simulink model "aero2_position_integral"  (R2024b)
settings: Solver=ode1  StartTime=0.0  StopTime=60  FixedStep=0.002  RelTol=1e-3
model workspace (MAT data in the model file):
  Dpos = 5.83392170192
  Dq = 3.88928113461
  Kaw = 20
  Kff = 1
  Ki = 1.84164606325
  Kint = 7.35390515018
  Kp = 0.216370391856
  Kpos = 11.344880808
  Kq = 3.78162693601
  Kref = 3.78162693601
  ReferenceRate = [0 0.002 0.004 0.006 0.008 0.01 0.012 0.014 0.016 0.018 0.02 0.022 ... (90003 elements, 30001x3)]
  U_h = timeseries
  U_h.Name = 'unnamed'
  U_h.DataInfo = tsdata.datametadata
  U_h.DataInfo.Interpolation = tsdata.interpolation
  U_h.DataInfo.Interpolation.Fhandle : function handle (value not decoded)
  U_h.DataInfo.Interpolation.Name = 'linear'
  U_h.TimeInfo = tsdata.timemetadata
  U_h.TimeInfo.Length = 30001
  U_h.TimeInfo.DuplicateTimes = 0
  U_h.TimeInfo.Time_ = [0 0.002 0.004 0.006 0.008 0.01 0.012 0.014 0.016 0.018 0.02 0.022 ... (30001 elements, 30001x1)]
  U_h.TimeInfo.Initialized = 1
  U_h.QualityInfo = tsdata.qualmetadata
  U_h.Data_ = [0 0 0 0 0 0 0 0 0 0 0 0 ... (30001 elements, 30001x1)]
  U_v = timeseries
  U_v.Name = 'unnamed'
  U_v.DataInfo = tsdata.datametadata
  U_v.DataInfo.Interpolation = tsdata.interpolation
  U_v.DataInfo.Interpolation.Fhandle : function handle (value not decoded)
  U_v.DataInfo.Interpolation.Name = 'linear'
  U_v.TimeInfo = tsdata.timemetadata
  U_v.TimeInfo.Length = 30001
  U_v.TimeInfo.DuplicateTimes = 0
  U_v.TimeInfo.Time_ = [0 0.002 0.004 0.006 0.008 0.01 0.012 0.014 0.016 0.018 0.02 0.022 ... (30001 elements, 30001x1)]
  U_v.TimeInfo.Initialized = 1
  U_v.QualityInfo = tsdata.qualmetadata
  U_v.Data_ = [0 0 0 0 0 0 0 0 0 0 0 0 ... (30001 elements, 30001x1)]
  X0 = [0; 0; 0; 0]
  meas_on = 0
(part 1 of 2)
settings Model: Creator=matiasgarcia  LastModifiedBy=matiasgarcia
settings DataIOCC: SaveOutput=off  SignalLogging=off  SaveTime=off

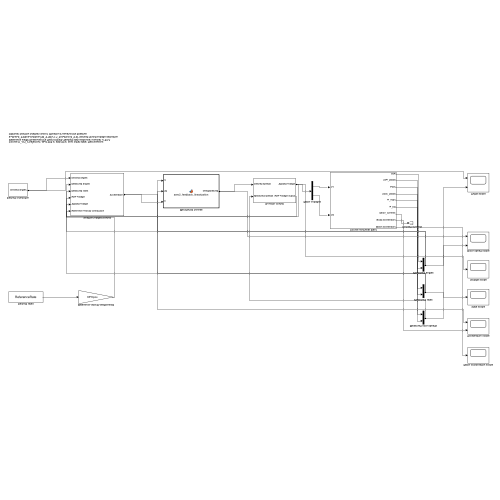
[thumbnail: Simulink's stored preview of the top-level diagram]
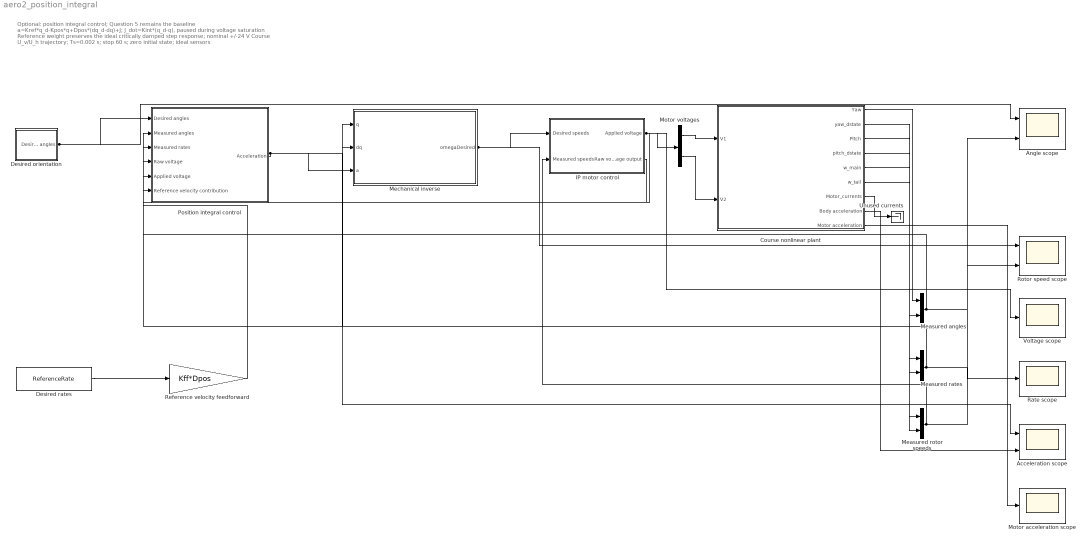
== system aero2_position_integral ==
  note: Optional: position integral control; Question 5 remains the baseline
      | a=Kref*q_d-Kpos*q+Dpos*(dq_d-dq)+J; J_dot=Kint*(q_d-q), paused during voltage saturation
      | Reference weight preserves the ideal critically damped step response; nominal +/-24 V
      | Course U_v/U_h trajectory; Ts=0.002 s; stop 60 s; zero initial state; ideal sensors
  Acceleration scope : Scope  NumInputPorts=2
  Angle scope : Scope  NumInputPorts=2
  Course nonlinear plant : Subsystem  mask{meas=meas_on}
      mask prompts: meas "Measurement effects (1 = encoder quantization + sensor noise, 0 = ideal)"
      mask help: Simplified twin-rotor model (eq. (simp) of twin_rotor_FL_merged.tex) with DC-motor rotor dynamics. Inputs: V1 main-rotor voltage, V2 tail-rotor voltage [V]. Outputs: same signals as the QUARC interface of lin_feedback_v1.slx, continuous (no zero-order holds; sensor noise generated at Ts).
  Desired orientation : Subsystem
  Desired rates : FromWorkspace  VariableName=ReferenceRate  OutputAfterFinalValue=Holding final value
  IP motor control : Subsystem
  Measured angles : Mux  Inputs=2
  Measured rates : Mux  Inputs=2
  Measured rotor speeds : Mux  Inputs=2
  Mechanical inverse : MATLAB Function  TreatAsAtomicUnit=on
  Motor acceleration scope : Scope
  Motor voltages : Demux  Outputs=2
  Position integral control : Subsystem
  Rate scope : Scope
  Reference velocity feedforward : Gain  Gain=Kff*Dpos
  Rotor speed scope : Scope  NumInputPorts=2
  Unused currents : Terminator
  Voltage scope : Scope
  wires:
  Measured angles/1 -> Position integral control/2(Measured angles), Mechanical inverse/1(q), Angle scope/2
  Measured rates/1 -> Position integral control/3(Measured rates), Mechanical inverse/2(dq), Rate scope/1
  IP motor control/2(Raw voltage output) -> Position integral control/4(Raw voltage)
  IP motor control/1(Applied voltage) -> Position integral control/5(Applied voltage), Motor voltages/1, Voltage scope/1
  Position integral control/1(Acceleration) -> Mechanical inverse/3(a), Acceleration scope/1
  Mechanical inverse/1(omegaDesired) -> IP motor control/1(Desired speeds), Rotor speed scope/1
  Measured rotor speeds/1 -> IP motor control/2(Measured speeds), Rotor speed scope/2
  Motor voltages/1 -> Course nonlinear plant/1(V1)
  Course nonlinear plant/1(Yaw) -> Measured angles/1
  Course nonlinear plant/2(yaw_dstate) -> Measured rates/1
  Course nonlinear plant/5(w_main) -> Measured rotor speeds/1
  Motor voltages/2 -> Course nonlinear plant/2(V2)
  Course nonlinear plant/3(Pitch) -> Measured angles/2
  Course nonlinear plant/4(pitch_dstate) -> Measured rates/2
  Course nonlinear plant/6(w_tail) -> Measured rotor speeds/2
  Course nonlinear plant/7(Motor_currents) -> Unused currents/1
  Course nonlinear plant/8(Body acceleration) -> Acceleration scope/2
  Course nonlinear plant/9(Motor acceleration) -> Motor acceleration scope/1
  Desired orientation/1(Desired angles) -> Position integral control/1(Desired angles), Angle scope/1
  Desired rates/1 -> Reference velocity feedforward/1
  Reference velocity feedforward/1 -> Position integral control/6(Reference velocity contribution)
